simulink model "week07_wheel_model"  (R2026a)
settings: Solver=ode45  StopTime=0.6  MaxStep=wheel.Ts/10  RelTol=1e-6  AbsTol=1e-9
model workspace (MAT data in the model file):
  referenceSpeed = 0.1
  stepTime = 0.2
  wheel.L = 0.0033
  wheel.R = 2.86
  wheel.Kt = 0.00798
  wheel.Kb = 0.00798
  wheel.J = 5.46e-06
  wheel.D = 3.38e-06
  wheel.gear = 9.68
  wheel.wheelRadius = 0.03
  wheel.Kp = 0.27509955055
  wheel.Ki = 3.89290939082
  wheel.Kd = 0
  wheel.Tf = 0
  wheel.Ts = 0.001
  wheel.voltageLimit = 9
values from neighbouring files (symbols this model uses):
  wheel = struct('L', L, 'R', R, 'Kt', Kt, 'Kb', Kb, 'J', J, 'D', D,      'gear', gear, 'wheelRadius', wheelRadius,      'Kp', C.Kp, 'Ki', C.Ki, 'Kd', C.Kd, 'Tf', C.Tf,      'Ts', Ts, 'voltageLimit', voltageLimit)    [PID_tune_v4.m]    (also in week07_pid_tune.m = struct('L', L, 'R', R, 'Kt', Kt, 'Kb', Kb, 'J', J, 'D', D,  )
libraries: slpidlib x1
settings Model: Creator=michaeljohansen  LastModifiedBy=michaeljohansen

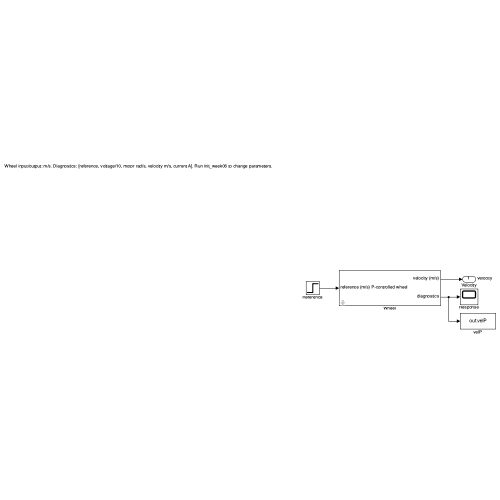
[thumbnail: Simulink's stored preview of the top-level diagram]
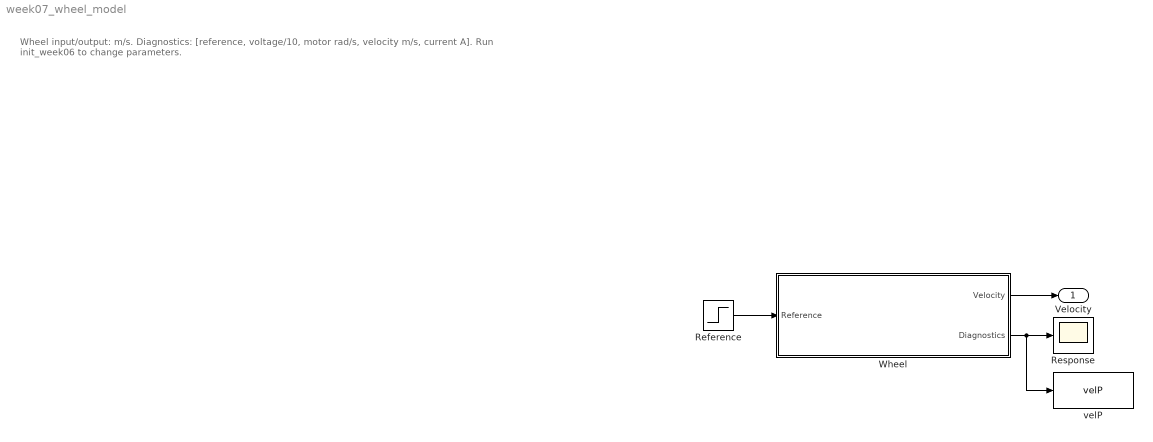
== system week07_wheel_model ==
  note: Wheel input/output: m/s. Diagnostics: [reference, voltage/10, motor rad/s, velocity m/s, current A]. Run init_week06 to change parameters.
  Reference : Step  Time=stepTime  FinalValue=referenceSpeed  SampleTime=0
  Response : Scope
  Wheel : Subsystem  mask{L=wheel.L, R=wheel.R, Kt=wheel.Kt, Kb=wheel.Kb, J=wheel.J, D=wheel.D, gear=wheel.gear, wheelRadius=wheel.wheelRadius, Kp=wheel.Kp, Ts=wheel.Ts, voltageLimit=wheel.voltageLimit}
      mask Display: disp('P-controlled wheel'); port_label('input',1,'reference (m/s)'); port_label('output',1,'velocity (m/s)'); port_label('output',2,'diagnostics');
  velP : ToWorkspace  VariableName=velP  SaveFormat=Timeseries  SampleTime=-1
  Velocity : Outport  SignalName=Velocity
  wires:
  Reference/1 -> Wheel/1(Reference)
  Wheel/1(Velocity) -> Velocity/1
  Wheel/2(Diagnostics) -> Response/1, velP/1

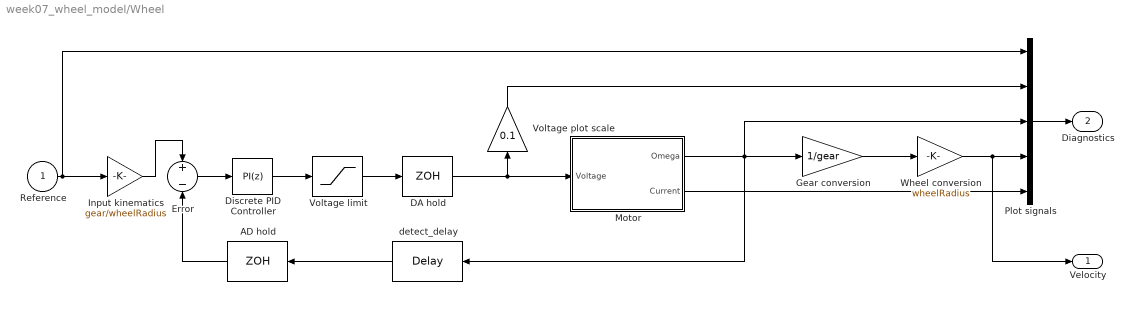
== system week07_wheel_model/Wheel ==
  Reference : Inport
  AD hold : ZeroOrderHold  SampleTime=Ts
  DA hold : ZeroOrderHold  SampleTime=Ts
  Discrete PID Controller : slpidlib/PID Controller  Controller=PI  Form=Parallel  TimeDomain=Discrete-time  UseExternalTs=off  SampleTime=Ts  IntegratorMethod=Forward Euler  FilterMethod=Backward Euler  ControllerParametersSource=internal  P=wheel.Kp  I=wheel.Ki  UseKiTs=off  D=wheel.Kd  UseExternalDerivativeSource=off  N=1/wheel.Tf  UseFilter=on  TunerSelectOption=Transfer Function Based (PID Tuner App)  InitialConditionSource=internal  InitialConditionForIntegrator=0  InitialConditionForFilter=0  DifferentiatorICPrevScaledInput=0  ExternalReset=none  TrackingMode=off  Kt=1  LimitOutput=on  SatLimitsSource=internal  UpperSaturationLimit=9  LowerSaturationLimit=-9  LinearizeAsGain=off  AntiWindupMode=clamping  Kb=1  LimitIntegrator=off  UpperIntegratorSaturationLimit=inf  LowerIntegratorSaturationLimit=-inf  POutMin=[]  POutMax=[]  IOutMin=[]  IOutMax=[]  DOutMin=[]  DOutMax=[]  NOutMin=[]  NOutMax=[]  SumOutMin=[]  SumOutMax=[]  SaturationOutMin=[]  SaturationOutMax=[]  PParamMin=[]  PParamMax=[]  IParamMin=[]  IParamMax=[]  DParamMin=[]  DParamMax=[]  NParamMin=[]  NParamMax=[]  KbParamMin=[]  KbParamMax=[]  KtParamMin=[]  KtParamMax=[]  KbOutMin=[]  KbOutMax=[]  KtOutMin=[]  KtOutMax=[]  IntegratorOutMin=[]  IntegratorOutMax=[]  FilterOutMin=[]  FilterOutMax=[]  SumI1OutMin=[]  SumI1OutMax=[]  SumI2OutMin=[]  SumI2OutMax=[]  SumI3OutMin=[]  SumI3OutMax=[]  SumI4OutMin=[]  SumI4OutMax=[]  SumDOutMin=[]  SumDOutMax=[]  DifferentiatorOutMin=[]  DifferentiatorOutMax=[]  FilterDiffOutCoefMin=[]  FilterDiffOutCoefMax=[]  ReciprocalOutMin=[]  ReciprocalOutMax=[]  SumDenOutMin=[]  SumDenOutMax=[]  SumNumOutMin=[]  SumNumOutMax=[]  DivideOutMin=[]  DivideOutMax=[]  UdiffTsProdOutMin=[]  UdiffTsProdOutMax=[]  NTsProdOutMin=[]  NTsProdOutMax=[]  UintegralTsProdOutMin=[]  UintegralTsProdOutMax=[]  UngainTsProdOutMin=[]  UngainTsProdOutMax=[]  ClampingZeroOutDataTypeStr=Inherit: Inherit via back propagation  ClampingZeroOutMin=[]  ClampingZeroOutMax=[]  FilterDenConstantOutDataTypeStr=Inherit: Inherit via back propagation  FilterDenConstantOutMin=[]  FilterDenConstantOutMax=[]  PCopyOutDataTypeStr=Inherit: Inherit via back propagation  PCopyOutMin=[]  PCopyOutMax=[]  NCopyOutDataTypeStr=Inherit: Inherit via back propagation  NCopyOutMin=[]  NCopyOutMax=[]  IntegratorContinuousStateAttributes=''  IntegratorStateMustResolveToSignalObject=off  IntegratorRTWStateStorageClass=Auto  FilterContinuousStateAttributes=''  FilterStateMustResolveToSignalObject=off  FilterRTWStateStorageClass=Auto  ParallelPVariant=InternalParameters  IdealPVariant=Disabled  IVariant=InternalParameters  DVariant=Disabled  IntegratorVariant=Discrete  SatVariant=Enabled  AWVariant=DiscClampingParallel  PCopyVariant=Disabled  TRVariant=Disabled  FdbkBlocksVariant=Forward  IdealPFdbkVariant=Disabled  SatFdbkVariant=Disabled  DerivativeFilterVariant=Disabled  NVariant=Disabled  NCopyVariant=Disabled_SignalSpec  FilterICVariant=Disabled  IntegratorICVariant=InternalICs  ExternalResetVariant=Disabled  TRSumVariant=Passthrough  SumFdbkVariant=Disabled  SumVariant=Sum_PI  TsampFilterVariant=InternalTs  TsampNgainVariant=Passthrough  TsampIntegralVariant=Disabled_SignalSpec  ExternalSaturationOutDataTypeStr=Inherit: Same as second input  DerivativeSourceVariant=Disabled  PreIntVariant=InternalPreInt
      settings: LibrarySourceBlock=simulink/Discrete/Discrete PID Controller
  Error : Sum  Inputs=+-
  Gear conversion : Gain  Gain=1/gear
  Input kinematics : Gain  Gain=gear/wheelRadius
  Motor : Subsystem
  Plot signals : Mux  Inputs=5
  Voltage limit : Saturate  UpperLimit=voltageLimit  LowerLimit=-voltageLimit
  Voltage plot scale : Gain  Gain=0.1
  Wheel conversion : Gain  Gain=wheelRadius
  detect_delay : TransportDelay  DelayTime=Ts
  Velocity : Outport
  Diagnostics : Outport  Port=2
  wires:
  Plot signals/1 -> Diagnostics/1
  Reference/1 -> Plot signals/1, Input kinematics/1
  Motor/2(Current) -> Plot signals/5
  Wheel conversion/1 -> Velocity/1, Plot signals/4
  Motor/1(Omega) -> detect_delay/1, Gear conversion/1, Plot signals/3
  Voltage limit/1 -> DA hold/1
  detect_delay/1 -> AD hold/1
  Input kinematics/1 -> Error/1
  Gear conversion/1 -> Wheel conversion/1
  AD hold/1 -> Error/2
  DA hold/1 -> Motor/1(Voltage), Voltage plot scale/1
  Voltage plot scale/1 -> Plot signals/2
  Error/1 -> Discrete PID Controller/1
  Discrete PID Controller/1 -> Voltage limit/1

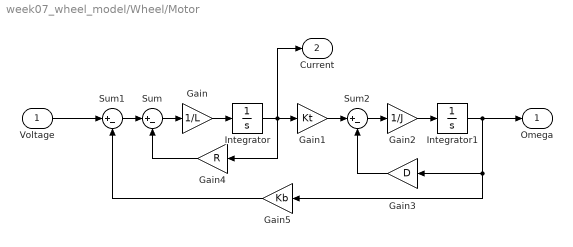
== system week07_wheel_model/Wheel/Motor ==
  Voltage : Inport
  Gain : Gain  Gain=1/L
  Gain1 : Gain  Gain=Kt
  Gain2 : Gain  Gain=1/J
  Gain3 : Gain  Gain=D
  Gain4 : Gain  Gain=R
  Gain5 : Gain  Gain=Kb
  Integrator : Integrator
  Integrator1 : Integrator
  Sum : Sum  Inputs=|+-
  Sum1 : Sum  Inputs=|+-
  Sum2 : Sum  Inputs=|+-
  Omega : Outport
  Current : Outport  Port=2
  wires:
  Voltage/1 -> Sum1/1
  Sum1/1 -> Sum/1
  Sum/1 -> Gain/1
  Gain/1 -> Integrator/1
  Integrator/1 -> Gain1/1, Gain4/1, Current/1
  Gain4/1 -> Sum/2
  Gain1/1 -> Sum2/1
  Sum2/1 -> Gain2/1
  Gain2/1 -> Integrator1/1
  Integrator1/1 -> Gain3/1, Gain5/1, Omega/1
  Gain3/1 -> Sum2/2
  Gain5/1 -> Sum1/2
